simulink model "Boost_Umbral_Dinamico"  (R2025b)
settings: Solver=ode4  StartTime=0.0  StopTime=0.6  FixedStep=2e-6  RelTol=1e-3
values from neighbouring files (symbols this model uses):
  J_min = 0.02    [Ejecutar_Punto1_Ruido_30Corridas.m]    (also in Ejecutar_Punto2_Analisis_Enmascaramiento.m; Ejecutar_Punto3_Comparacion_Adaptativos.m)
  k_sens = 4    [Ejecutar_Punto1_Ruido_30Corridas.m]
  N_ventana = 10000    [Ejecutar_Punto1_Ruido_30Corridas.m]
  x0 = [iL_ref; vc_ref]    [Parametros_Convertidor_Boost.m]
  xhat0 = [iL_ref; vc_ref]    [Parametros_Convertidor_Boost.m]
settings Model: Creator=ASUSTUF  LastModifiedBy=ASUSTUF

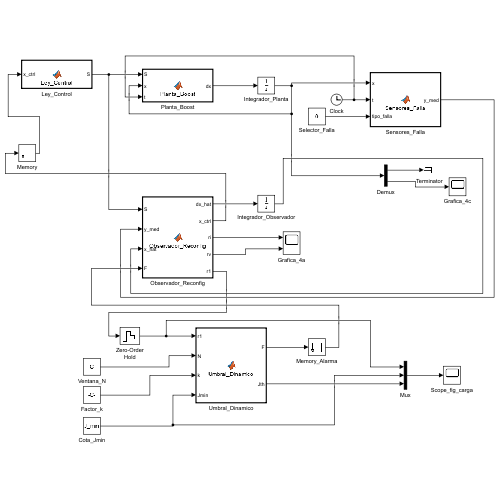
[thumbnail: Simulink's stored preview of the top-level diagram]
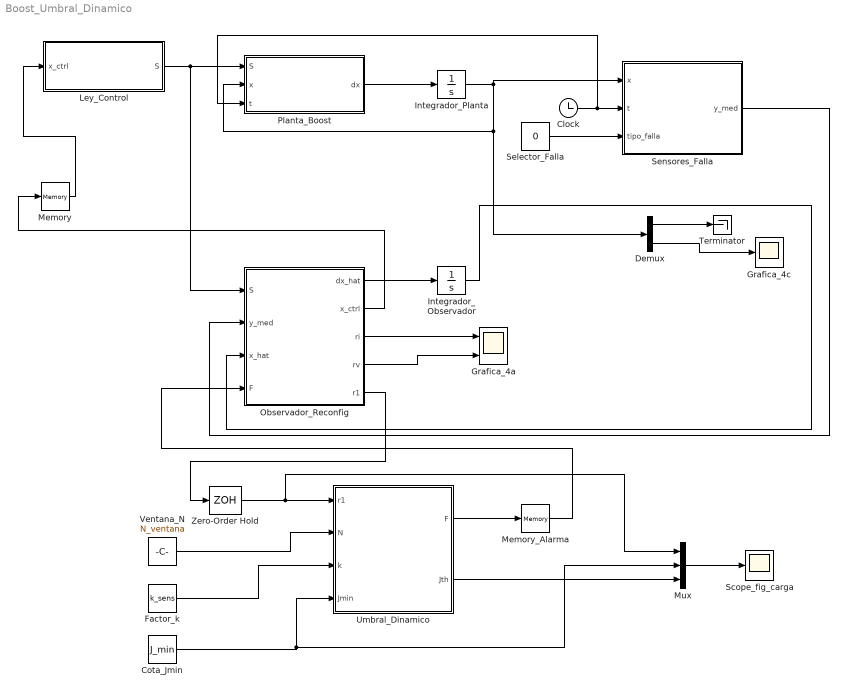
== system Boost_Umbral_Dinamico ==
  Clock : Clock
  Cota_Jmin : Constant  Value=J_min
  Demux : Demux  Outputs=2
  Factor_k : Constant  Value=k_sens
  Grafica_4a : Scope  NumInputPorts=2
      settings: ActiveDisplayYMinimum=-10.76281971037826  ActiveDisplayYMaximum=6.8965764434996784
  Grafica_4c : Scope
      settings: ActiveDisplayYMinimum=-1  ActiveDisplayYMaximum=1  DataLoggingVariableName=ScopeData2
  Integrador_Observador : Integrator  InitialCondition=xhat0
  Integrador_Planta : Integrator  InitialCondition=x0
  Ley_Control : MATLAB Function  TreatAsAtomicUnit=on
  Memory : Memory  InitialCondition=x0
  Memory_Alarma : Memory
  Mux : Mux  Inputs=3
  Observador_Reconfig : MATLAB Function  TreatAsAtomicUnit=on
  Planta_Boost : MATLAB Function  TreatAsAtomicUnit=on
  Scope_fig_carga : Scope
      settings: ActiveDisplayYMinimum=-0.062232102639306175  ActiveDisplayYMaximum=0.2084133455967464
  Selector_Falla : Constant  Value=0
  Sensores_Falla : MATLAB Function  TreatAsAtomicUnit=on
  Terminator : Terminator
  Umbral_Dinamico : MATLAB Function  TreatAsAtomicUnit=on
  Ventana_N : Constant  Value=N_ventana
  Zero-Order Hold : ZeroOrderHold  SampleTime=2e-6
  wires:
  Ley_Control/1(S) -> Observador_Reconfig/1(S), Planta_Boost/1(S)
  Planta_Boost/1(dx) -> Integrador_Planta/1
  Integrador_Planta/1 -> Sensores_Falla/1(x), Demux/1, Planta_Boost/2(x)
  Clock/1 -> Planta_Boost/3(t), Sensores_Falla/2(t)
  Selector_Falla/1 -> Sensores_Falla/3(tipo_falla)
  Sensores_Falla/1(y_med) -> Observador_Reconfig/2(y_med)
  Observador_Reconfig/1(dx_hat) -> Integrador_Observador/1
  Integrador_Observador/1 -> Observador_Reconfig/3(x_hat)
  Observador_Reconfig/3(ri) -> Grafica_4a/1
  Observador_Reconfig/4(rv) -> Grafica_4a/2
  Demux/2 -> Grafica_4c/1
  Demux/1 -> Terminator/1
  Observador_Reconfig/2(x_ctrl) -> Memory/1
  Memory/1 -> Ley_Control/1(x_ctrl)
  Observador_Reconfig/5(r1) -> Zero-Order Hold/1
  Zero-Order Hold/1 -> Mux/1, Umbral_Dinamico/1(r1)
  Ventana_N/1 -> Umbral_Dinamico/2(N)
  Factor_k/1 -> Umbral_Dinamico/3(k)
  Cota_Jmin/1 -> Mux/2, Umbral_Dinamico/4(Jmin)
  Umbral_Dinamico/1(F) -> Memory_Alarma/1
  Memory_Alarma/1 -> Observador_Reconfig/4(F)
  Umbral_Dinamico/2(Jth) -> Mux/3
  Mux/1 -> Scope_fig_carga/1

== matlab function Boost_Umbral_Dinamico/Planta_Boost ==
  data: S input; dx output; x input; t input
function dx = Planta_Boost(S, x, t)
Vin = 190;
C0  = 0.00285;
L   = 0.005;
R   = 0.082;

% Experimento A: Perturbación transitoria de carga de 3.5% (100 a 96.6 Ohms) en t = 0.3 s
if t >= 0.3
    tau = t - 0.3;
    if tau <= 0.040
        pulso = tau / 0.040;
    else
        pulso = exp(-(tau - 0.040) / 0.025);
    end
    Rload = 100 / (1 + 0.035 * pulso);
else
    Rload = 100;
end

A0 = [-R/L, -1/L; 1/C0, -1/(Rload*C0)];
A1 = [-R/L,  0;   0,    -1/(Rload*C0)];
B  = [1/L; 0];

if S == 0
    dx = A0 * x + B * Vin;
else
    dx = A1 * x + B * Vin;
end
end

== matlab function Boost_Umbral_Dinamico/Ley_Control ==
  data: x_ctrl input; S output
function S = Ley_Control(x_ctrl)
% Parámetros desde las ecuaciones del artículo
Vin   = 190;
C0    = 0.00285;
L     = 0.005;
R     = 0.082;
Rload = 100;

x_star = [7.6; 380];
P_lyap = [L, 0; 0, C0];

A0 = [-R/L, -1/L; 1/C0, -1/(Rload*C0)];
A1 = [-R/L,  0;   0,    -1/(Rload*C0)];
B  = [1/L; 0];

% Error de estado z = x - x*
z = x_ctrl - x_star;

% Derivadas de la función de Lyapunov V_dot para S=0 y S=1
V0_dot = 2 * z' * P_lyap * (A0 * x_ctrl + B * Vin);
V1_dot = 2 * z' * P_lyap * (A1 * x_ctrl + B * Vin);

% Regla de conmutación: elegir el modo con menor derivada
if V0_dot < V1_dot
    S = 0;
else
    S = 1;
end
end

== matlab function Boost_Umbral_Dinamico/Sensores_Falla ==
  data: x input; y_med output; t input; tipo_falla input
function y_med = Sensores_Falla(x, t, tipo_falla)
% x(1) = i_L, x(2) = v_c
% tipo_falla = 1 -> Circuito abierto en sensor de corriente (Fig. 4a, 4b, 4c)
% tipo_falla = 2 -> Circuito abierto en sensor de voltaje   (Fig. 4d, 4e, 4f)

y_med = x;

if t >= 0.2
    if tipo_falla == 1
        y_med(1) = 0; % Sensor de corriente en circuito abierto (f_i = -i_L)
    elseif tipo_falla == 2
        y_med(2) = 0; % Sensor de voltaje en circuito abierto (f_v = -v_c)
    end
end
end

== matlab function Boost_Umbral_Dinamico/Observador_Reconfig ==
  data: S input; dx_hat output; y_med input; x_hat input; x_ctrl output; ri output; rv output; r1 output; F input
function [dx_hat, x_ctrl, ri, rv, r1] = Observador_Reconfig(S, y_med, x_hat, F)
Vin   = 190;
C0    = 0.00285;
L     = 0.005;
R     = 0.082;
Rload = 100; % El observador conserva el Rload nominal de 100 Ohms

x_star = [7.6; 380];

H = [36.4677, -17.0967; 
     28.5219,  75.6359];

A0 = [-R/L, -1/L; 1/C0, -1/(Rload*C0)];
A1 = [-R/L,  0;   0,    -1/(Rload*C0)];
B  = [1/L; 0];

if S == 0
    A_s = A0;
else
    A_s = A1;
end

% 1. Generación de residuos
y_hat = x_hat;
r = y_med - y_hat;
ri = r(1);
rv = r(2);
r1 = ri^2 + rv^2;

% 2. Reconfiguración activada por la señal F del Umbral Dinámico
if F > 0.5
    x_ctrl = x_hat;
    dx_hat = A_s * x_hat + B * Vin + H * (x_star - y_hat);
else
    x_ctrl = y_med;
    dx_hat = A_s * x_hat + B * Vin + H * (y_med - y_hat);
end
end

== matlab function Boost_Umbral_Dinamico/Umbral_Dinamico ==
  data: r1 input; F output; N input; k input; Jmin input; Jth output
function [F, Jth] = Umbral_Dinamico(r1, N, k, Jmin)
% Umbral dinámico con ventana móvil y cota inferior (Anexo A optimizado)
% r1: residuo r_i^2 + r_v^2; N: ventana en muestras (10000 a 25000);
% k: factor de sensibilidad (3, 4, 5); Jmin: cota inferior (0.02).

NMAX = 25000; % Soporta ventanas de hasta 50 ms con paso de 2 us
persistent buf idx cnt sum_r1 sum_r2
if isempty(buf)
    buf = zeros(NMAX, 1);
    idx = 1;
    cnt = 0;
    sum_r1 = 0;
    sum_r2 = 0;
end

% Limitar N por seguridad al tamaño máximo del buffer
N_eff = min(max(round(N), 1), NMAX);

% 1. Calcular media (m) y desviación estándar (s) solo con muestras pasadas
if cnt > 0
    m = sum_r1 / cnt;
    varianza = (sum_r2 / cnt) - (m^2);
    s = sqrt(max(varianza, 0));
else
    m = 0;
    s = 0;
end

% 2. Evaluar umbral dinámico y condición de alarma (Salidas tipo double)
Jth = max(Jmin, m + k * s);
F   = double(r1 > Jth);

% 3. Regla del buffer: actualizar solo cuando NO hay alarma (F == 0)
if F == 0
    if cnt == N_eff
        % Restar la muestra más antigua que sale de la ventana circular
        old_val = buf(idx);
        sum_r1 = sum_r1 - old_val;
        sum_r2 = sum_r2 - (old_val^2);
    else
        cnt = cnt + 1;
    end
    % Guardar la muestra actual y acumular sumas
    buf(idx) = r1;
    sum_r1 = sum_r1 + r1;
    sum_r2 = sum_r2 + (r1^2);
    idx = mod(idx, N_eff) + 1;
end
end
